simulink model "TCLab_Implementation"  (R2026a)
settings: Solver=FixedStepDiscrete  StopTime=inf  FixedStep=1  EnableMultiTasking=on
undefined symbols (not defined in the file): T_ref, Ts
libraries: arduinolib x2, dspstat3 x1
settings Model: SILPILModeSetting=veronly  ExtModeTrigDuration=2  Creator=jordy  LastModifiedBy=jordy
settings HardwareCC: ProdBitPerInt=16.0  ProdBitPerPointer=16.0  ProdBitPerSizeT=16.0  ProdBitPerPtrDiffT=16.0  ProdWordSize=8.0  ProdHWDeviceType=Atmel->AVR
settings RTWCC: SystemTargetFile=ert.tlc  HardwareBoard=Arduino Leonardo  TLCOptions=-aInlineSetEventsForThisBaseRateFcn=TLC_FALSE -aSuppressMultiTaskScheduler=TLC_FALSE -aRateBasedStepFcn=1  Toolchain=Arduino AVR  BuildConfiguration=Faster Runs  Description=Embedded Coder
settings ERTTargetCC: ExtModeTransport=3.0  ExtModeAutomaticAllocSize=off  ExtModeStaticAllocSize=250.0  SupportContinuousTime=on  SupportVariableSizeSignals=on

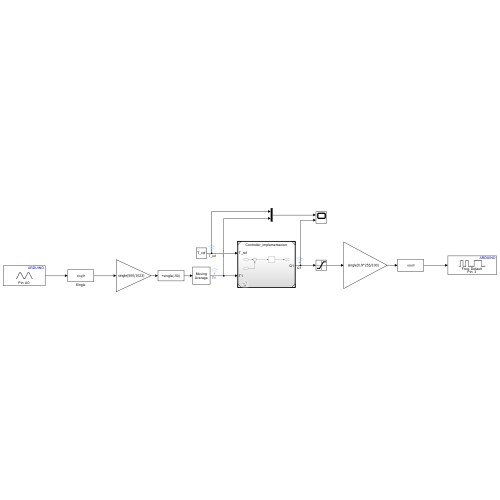
[thumbnail: Simulink's stored preview of the top-level diagram]
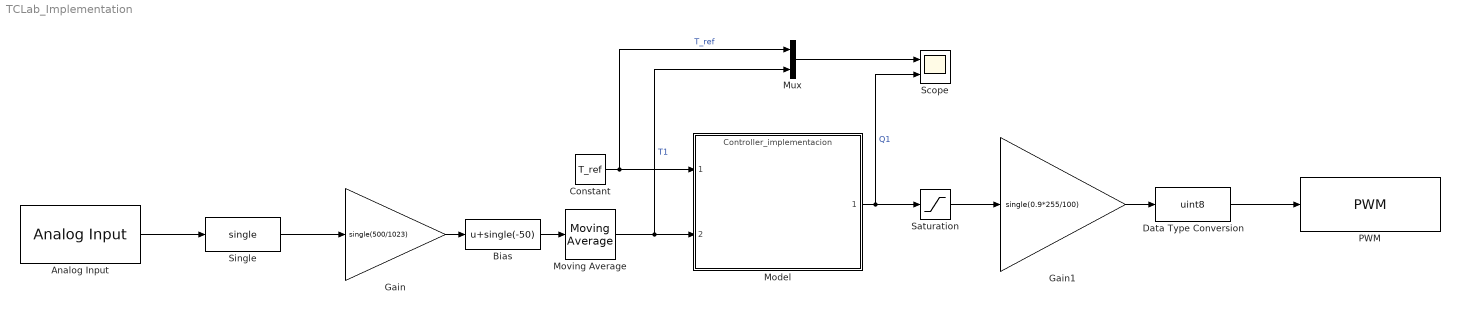
== system TCLab_Implementation ==
  Analog Input : arduinolib/Analog Input  pinNumber=0  ReadResultsOnly=off  ConversionTriggerSource=Software  ExternalTriggerType=uint32( 0 )  OutputDataType=uint16  EnableConversionCompleteNotify=off  EnableOuputStatus=off  SampleTime=Ts  blockPlatform=arduino
      settings: LibrarySourceBlock=gizmoLibrary/Arduino Utilities/Analog Input
  Bias : Bias  Bias=single(-50)  SaturateOnIntegerOverflow=off
  Constant : Constant  Value=T_ref  OutDataTypeStr=single
  Data Type Conversion : DataTypeConversion  OutDataTypeStr=uint8  SaturateOnIntegerOverflow=off  RndMeth=Floor
  Gain : Gain  Gain=single(500/1023)
  Gain1 : Gain  Gain=single(0.9*255/100)
  Model : ModelReference  ModelNameDialog=Controller_implementacion  SimulationMode=Normal  ModelReferenceVersion=1.27
  Moving Average : dspstat3/Moving Average  Method=Exponential weighting  ForgettingFactorPort=off  SpecifyWindowLength=on  WindowLengthSource=Property  MaxWindowLength=20  WindowLength=4  OverlapLength=3  AllowArbitraryInputLength=off  ForgettingFactor=single(0.5)  SimulateUsing=Code generation
  Mux : Mux  Inputs=2
  PWM : arduinolib/PWM  pinNumber=3  frequencyType=Default  desiredFrequency=50  achievableFrequency=50
      settings: LibrarySourceBlock=gizmoLibrary/Arduino Utilities/PWM
  Saturation : Saturate  UpperLimit=90  LowerLimit=0
  Scope : Scope  NumInputPorts=2
      settings: TimeSpan=600
  Single : DataTypeConversion  OutDataTypeStr=single  SaturateOnIntegerOverflow=off  RndMeth=Floor
  wires:
  Analog Input/1 -> Single/1
  Single/1 -> Gain/1
  Gain/1 -> Bias/1
  Bias/1 -> Moving Average/1
  Moving Average/1 -> Mux/2, Model/2  "T1"
  Constant/1 -> Mux/1, Model/1  "T_ref"
  Model/1 -> Scope/2, Saturation/1  "Q1"
  Saturation/1 -> Gain1/1
  Gain1/1 -> Data Type Conversion/1
  Data Type Conversion/1 -> PWM/1
  Mux/1 -> Scope/1
